simulink model "planta_PROTEC_fornalha_LC"  (Simulink 8.8)
settings: Solver=ode3  StartTime=0.0  StopTime=800  FixedStep=tempo_amostragem  MaxStep=1e1  MinStep=1e-2  EnableMultiTasking=on
InitFcn:
  | planta_PROTEC_inicializacao
values from neighbouring files (symbols this model uses):
  Estado_Estacionario = [2 38.1987406965 21.9709981215 1.00092553605 3.07737941356 1.5 0.843438999559 0.0384242731301 0.118136727311 1.3 0.304251987406 0.577644341688 ... (188 elements, 1x188)]    [planta_PROTEC_estado_estacionario_inicial.mat]
  tempo_amostragem = 1e-2    (= 0.01)    [planta_PROTEC_inicializacao.m]
libraries: simulink_extras x6
(part 3 of 3)

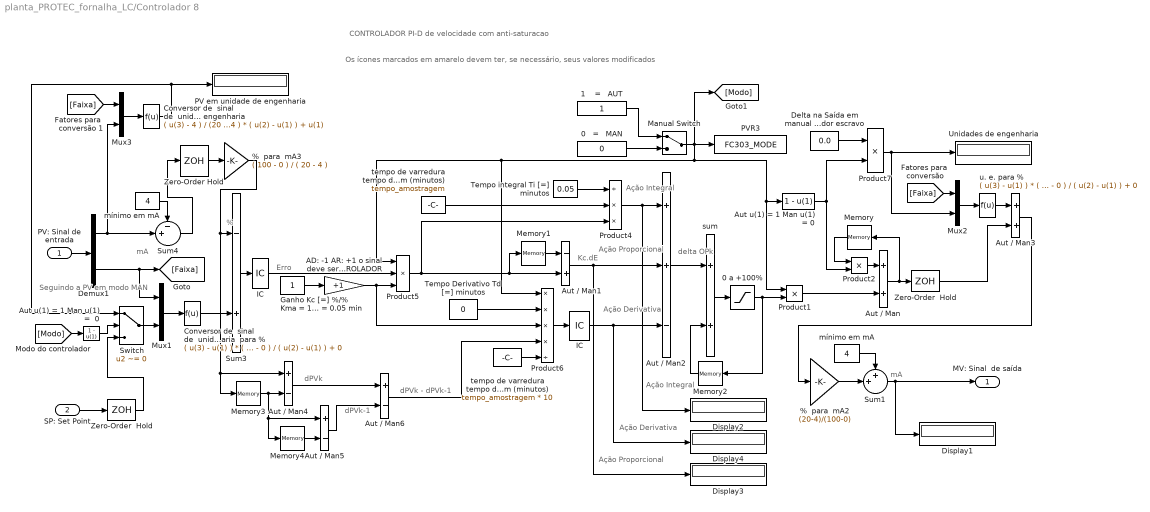
== system planta_PROTEC_fornalha_LC/Controlador 8 ==
  note: Ação
      | Derivativa
  note: dPVk - dPVk-1
  note: dPVk
  note: dPVk-1
  note: delta
      | OPk
  note: Ação
      | Integral
  note: Ação
      | Proporcional
  note: Kc.dE
  note: %
  note: mA
  note: CONTROLADOR PI-D de velocidade com anti-saturacao
  note: Os ícones marcados em amarelo devem ter, se necessário, seus valores modificados
  note: Erro
  note: mA
  note: Ação
      | Integral
  note: Ação
      | Derivativa
  note: Ação
      | Proporcional
  note: Seguindo a PV
      | em modo MAN
  PV: Sinal de entrada : Inport
  SP: Set Point : Inport  Port=2
  "  1    =   AUT" : Constant
  " IC" : InitialCondition  Value=0
  %  para  mA2 : Gain  Gain=(20-4)/(100-0)  SaturateOnIntegerOverflow=on  OutDataTypeStr=Inherit: Same as input  ParamDataTypeStr=Inherit: Same as input
  %  para  mA3 : Gain  Gain=( 100 - 0 ) / ( 20 - 4 )  SaturateOnIntegerOverflow=on  OutDataTypeStr=Inherit: Same as input  ParamDataTypeStr=Inherit: Same as input
  0   =   MAN : Constant  Value=0
  0 a +100% : Saturate  UpperLimit=100  LowerLimit=0  LinearizeAsGain=off
  "AD: -1 AR: +1 o sinal deve ser modificado para a  correta  AÇÃO  DO  CONTROLADOR  " : Gain  Gain=+1  SaturateOnIntegerOverflow=on  OutDataTypeStr=Inherit: Same as input  ParamDataTypeStr=Inherit: Same as input
  Aut / Man : Sum  SaturateOnIntegerOverflow=on  InputSameDT=on  OutDataTypeStr=Inherit: Same as first input
  Aut / Man1 : Sum  Inputs=-+  SaturateOnIntegerOverflow=on  InputSameDT=on  OutDataTypeStr=Inherit: Same as first input
  Aut / Man2 : Sum  Inputs=++-  SaturateOnIntegerOverflow=on  InputSameDT=on  OutDataTypeStr=Inherit: Same as first input
  Aut / Man3 : Sum  SaturateOnIntegerOverflow=on  InputSameDT=on  OutDataTypeStr=Inherit: Same as first input
  Aut / Man4 : Sum  Inputs=+-  SaturateOnIntegerOverflow=on  InputSameDT=on  OutDataTypeStr=Inherit: Same as first input
  Aut / Man5 : Sum  Inputs=+-  SaturateOnIntegerOverflow=on  InputSameDT=on  OutDataTypeStr=Inherit: Same as first input
  Aut / Man6 : Sum  Inputs=+-  SaturateOnIntegerOverflow=on  InputSameDT=on  OutDataTypeStr=Inherit: Same as first input
  Aut u(1) = 1 Man u(1) =  0 : Fcn  Expr=1 - u(1)
  Aut u(1) = 1 Man u(1) = 0 : Fcn  Expr=1 - u(1)
  Conversor de  sinal de  unidades  de  engenharia  para % : Fcn  Expr=( u(3) - u(1) ) * ( 100 - 0 ) / ( u(2) - u(1) ) + 0
  Conversor de  sinal de  unidades  de  mA  para  engenharia : Fcn  Expr=( u(3) - 4 ) / (20 - 4 ) * ( u(2) - u(1) ) + u(1)
  Delta na Saída em manual do controlador [=] unidades de engenharia do SP do controlador escravo : Constant  Value=0.0
  Demux1 : Demux  Outputs=[ 1 2 ]
  Display{1..4} (4 alike) : Display
  Ganho Kc [=] %/% Kma = 1 mA/mA Lambda = 0.05 min : Constant
  IC : InitialCondition  Value=0
  Manual Switch : ManualSwitch
  Memory{,2..4} (4 alike) : Memory  X0=50  InheritSampleTime=on
  Memory1 : Memory  InheritSampleTime=on
  Mux1 : Mux  Inputs=[ 2 1 ]
  Mux2 : Mux  Inputs=[ 2 1 ]
  Mux3 : Mux  Inputs=[ 2 1 ]
  PV em unidade de engenharia : Display
  PVR3 : ToWorkspace  VariableName=FC303_MODE  SampleTime=-1
      settings: Decimation=10
  Product1 : Product  SaturateOnIntegerOverflow=on  RndMeth=Zero  InputSameDT=on  OutDataTypeStr=Inherit: Same as first input
  Product2 : Product  SaturateOnIntegerOverflow=on  RndMeth=Zero  InputSameDT=on  OutDataTypeStr=Inherit: Same as first input
  Product4 : Product  Inputs=/**  SaturateOnIntegerOverflow=on  RndMeth=Zero  InputSameDT=on  OutDataTypeStr=Inherit: Same as first input
  Product5 : Product  Inputs=3  SaturateOnIntegerOverflow=on  RndMeth=Zero  InputSameDT=on  OutDataTypeStr=Inherit: Same as first input
  Product6 : Product  Inputs=****/  SaturateOnIntegerOverflow=on  RndMeth=Zero  InputSameDT=on  OutDataTypeStr=Inherit: Same as first input
  Product7 : Product  SaturateOnIntegerOverflow=on  RndMeth=Zero  InputSameDT=on  OutDataTypeStr=Inherit: Same as first input
  Sum1 : Sum  Inputs=++|  SaturateOnIntegerOverflow=on  InputSameDT=on  OutDataTypeStr=Inherit: Same as first input
  Sum3 : Sum  Inputs=-+  SaturateOnIntegerOverflow=on  InputSameDT=on  OutDataTypeStr=Inherit: Same as first input
  Sum4 : Sum  Inputs=-+|  SaturateOnIntegerOverflow=on  InputSameDT=on  OutDataTypeStr=Inherit: Same as first input
  Switch : Switch  Criteria=u2 ~= 0  RndMeth=Nearest  SaturateOnIntegerOverflow=on
  Tempo Derivativo Td [=] minutos : Constant  Value=0
  Tempo integral Ti [=] minutos : Constant  Value=0.05
  Unidades de engenharia : Display
  Zero-Order  Hold : ZeroOrderHold  SampleTime=tempo_amostragem
  "Zero-Order  Hold " : ZeroOrderHold  SampleTime=tempo_amostragem
  "Zero-Order Hold " : ZeroOrderHold  SampleTime=tempo_amostragem
  mínimo em mA : Constant  Value=4
  "mínimo em mA " : Constant  Value=4
  sum : Sum  SaturateOnIntegerOverflow=on  InputSameDT=on  OutDataTypeStr=Inherit: Same as first input
  tempo de varredura tempo de amostragem (minutos) : Constant  Value=tempo_amostragem
  "tempo de varredura tempo de amostragem (minutos) " : Constant  Value=tempo_amostragem * 10
  u. e. para % : Fcn  Expr=( u(3) - u(1) ) * ( 100 - 0 ) / ( u(2) - u(1) ) + 0
  MV: Sinal  de saída : Outport
  wires:
  "AD: -1 AR: +1 o sinal deve ser modificado para a  correta  AÇÃO  DO  CONTROLADOR  "/1 -> Product5/3, Product6/3
  " IC"/1 -> Aut / Man2/3, Display4/1
  "tempo de varredura tempo de amostragem (minutos) "/1 -> Product6/5
  Aut / Man5/1 -> Aut / Man6/2
  Aut / Man4/1 -> Aut / Man6/1
  Conversor de  sinal de  unidades  de  engenharia  para %/1 -> Sum3/2
  Product6/1 -> " IC"/1
  Tempo Derivativo Td [=] minutos/1 -> Product6/2
  Aut / Man6/1 -> Product6/4
  Memory4/1 -> Aut / Man5/2
  Memory3/1 -> Aut / Man4/2, Aut / Man5/1, Memory4/1
  Ganho Kc [=] %/% Kma = 1 mA/mA Lambda = 0.05 min/1 -> "AD: -1 AR: +1 o sinal deve ser modificado para a  correta  AÇÃO  DO  CONTROLADOR  "/1
  IC/1 -> Product5/2
  0 a +100%/1 -> Product1/2, Memory2/1
  Memory2/1 -> sum/2
  sum/1 -> 0 a +100%/1
  Aut / Man2/1 -> sum/1
  Aut / Man1/1 -> Aut / Man2/2, Display3/1
  Product4/1 -> Aut / Man2/1, Display2/1
  Memory1/1 -> Aut / Man1/1
  Memory/1 -> Product2/1
  Aut / Man/1 -> Memory/1, Zero-Order  Hold/1
  Aut u(1) = 1 Man u(1) = 0/1 -> Product2/2, Product7/2
  Product2/1 -> Aut / Man/1
  Product1/1 -> Aut / Man/2
  Product5/1 -> Memory1/1, Aut / Man1/2, Product4/3
  Sum3/1 -> IC/1
  mínimo em mA/1 -> Sum4/1
  Demux1/1 -> Sum4/2, Mux3/2
  Mux1/1 -> Conversor de  sinal de  unidades  de  engenharia  para %/1
  SP: Set Point/1 -> "Zero-Order  Hold "/1
  PV: Sinal de entrada/1 -> Demux1/1
  "mínimo em mA "/1 -> Sum1/1
  Sum1/1 -> MV: Sinal  de saída/1, Display1/1
  Sum4/1 -> "Zero-Order Hold "/1
  "Zero-Order Hold "/1 -> %  para  mA3/1
  %  para  mA3/1 -> Memory3/1, Aut / Man4/1, Sum3/1
  Manual Switch/1 -> Aut u(1) = 1 Man u(1) = 0/1, Product1/1, Product5/1, Product6/1, [Modo], PVR3/1
  Delta na Saída em manual do controlador [=] unidades de engenharia do SP do controlador escravo/1 -> Product7/1
  Product7/1 -> Unidades de engenharia/1, Mux2/2
  Demux1/2 -> Mux1/1, [Faixa]
  "Zero-Order  Hold "/1 -> Switch/3
  u. e. para %/1 -> Aut / Man3/1
  Zero-Order  Hold/1 -> Aut / Man3/2
  Mux2/1 -> u. e. para %/1
  [Faixa] -> Mux2/1
  Aut / Man3/1 -> %  para  mA2/1
  %  para  mA2/1 -> Sum1/2
  "  1    =   AUT"/1 -> Manual Switch/1
  0   =   MAN/1 -> Manual Switch/2
  [Modo] -> Aut u(1) = 1 Man u(1) =  0/1
  Switch/1 -> Mux1/2
  Aut u(1) = 1 Man u(1) =  0/1 -> Switch/2
  Mux3/1 -> Conversor de  sinal de  unidades  de  mA  para  engenharia/1
  [Faixa] -> Mux3/1
  Conversor de  sinal de  unidades  de  mA  para  engenharia/1 -> Switch/1, PV em unidade de engenharia/1
  Tempo integral Ti [=] minutos/1 -> Product4/1
  tempo de varredura tempo de amostragem (minutos)/1 -> Product4/2

== system planta_PROTEC_fornalha_LC/Dados economicos da  Planta PROTEC1 ==
  note: Sugestões e críticas enviar para o autor:
      |
      | e-mail: kalid@ufba.br
      |
      | Departamento de Engenharia Química da UFBA
      | Tel: (71) 3283.9811  ou  (71) 9188.3316
      | Arquivos e outras informações em
      |
      | www.PEI.ufba.br
  note: INFORMAÇÕES  PARA  AVALIAÇÃO  ECONÔMICA  DA  PLANTA  PROTEC
      |
      | Preço de compra de A:                   prA =   1 000.xA^8             u.e./t de A
      | Preço de venda  de B:                    prB =  10 000.xB^0.5         u.e./t de produto, para xB >= 0.755
      |                                                        prB =    1 000.xB                u.e./t de produto, para xB < 0.755
      | Preço de compra do combustível:   prC =   3 000                     u.e./t de combustível
      | Preço do tratamento do efluente:    prE =   2 000                     u.e./t de efluente
      | Preço de venda  de vapor:              prV =      500.PV^2/18.52  u.e./t de produto
      | Preço do catalisador:                   prCat = 10 000/kg de catalisador
      | Custo de processamento:                ctP =     500.(Fp)^3          u.e./t de carga processada
      | O custo de processamento inclui todos os custos variaveis, exceto os explicitados anteriormente
      |
      | xA - fração molar de A na alimentação
      | xB - fração molar de B no produto
      | PV - Pressão do Vapor [=] kgf/cm²
      | Fp - vazão processada
      |
      | u.e. - unidade econômica

== system planta_PROTEC_fornalha_LC/E 1 ==
  note: Exaustor
  Sinal de entrada : Inport
  Sinal de saída : Outport
  wires:
  Sinal de entrada/1 -> Sinal de saída/1

== system planta_PROTEC_fornalha_LC/E 312 ==
  note: Exaustor
  Sinal de entrada : Inport
  Sinal de saída : Outport
  wires:
  Sinal de entrada/1 -> Sinal de saída/1

== system planta_PROTEC_fornalha_LC/FE 1 ==
  note: Placa de orifício
  note: F
  note: T
  In1 : Inport
  Demux26 : Demux  Outputs=2
  Terminator1 : Terminator
  Out1 : Outport
  Out2 : Outport  Port=2
  wires:
  Demux26/2 -> Terminator1/1
  Demux26/1 -> Out1/1
  In1/1 -> Demux26/1, Out2/1

== system planta_PROTEC_fornalha_LC/FE 2 ==
  note: x
  note: T
  note: F
  note: Placa de orifício
  In1 : Inport
  Demux26 : Demux  Outputs=3
  Terminator1 : Terminator
  Terminator9 : Terminator
  Out1 : Outport
  Out2 : Outport  Port=2
  wires:
  In1/1 -> Out2/1, Demux26/1
  Demux26/1 -> Out1/1
  Demux26/3 -> Terminator9/1
  Demux26/2 -> Terminator1/1

== system planta_PROTEC_fornalha_LC/FE 302 ==
  note: T
  note: F
  note: Placa de orifício
  In1 : Inport
  Demux26 : Demux  Outputs=2
  Terminator1 : Terminator
  Out1 : Outport
  Out2 : Outport  Port=2
  wires:
  In1/1 -> Out2/1, Demux26/1
  Demux26/1 -> Out1/1
  Demux26/2 -> Terminator1/1

== system planta_PROTEC_fornalha_LC/FE 303 ==
  note: Placa de orifício
  note: F
  note: T
  note: x
  In1 : Inport
  Demux26 : Demux  Outputs=3
  Terminator1 : Terminator
  Terminator9 : Terminator
  Out1 : Outport
  Out2 : Outport  Port=2
  wires:
  Demux26/2 -> Terminator1/1
  Demux26/3 -> Terminator9/1
  Demux26/1 -> Out1/1
  In1/1 -> Demux26/1, Out2/1

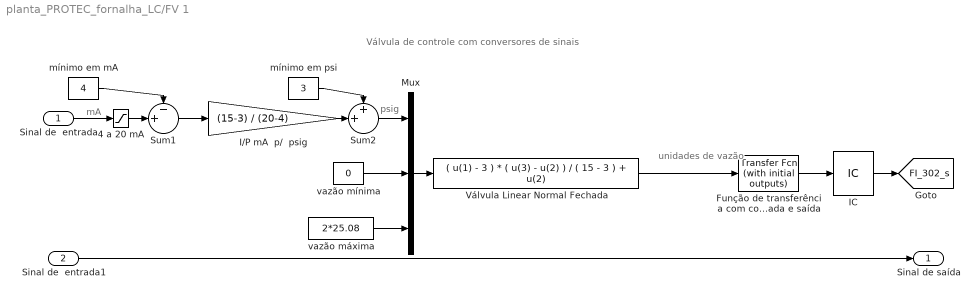
== system planta_PROTEC_fornalha_LC/FV 1 ==
  note: mA
  note: Válvula de controle com conversores de sinais
  note: unidades
      | de vazão
  note: psig
  Sinal de  entrada : Inport
  Sinal de  entrada1 : Inport  Port=2
  4 a 20 mA : Saturate  UpperLimit=20  LowerLimit=4
  Função de transferência com condição inicial  na entrada e saída : simulink_extras/Additional Linear/Transfer Fcn (with initial outputs)  N=[1]  D="[0.05   1 ]"  Y0=Estado_Estacionario(38)  U0=Estado_Estacionario(38)
  I/P mA  p/  psig : Gain  Gain=(15-3) / (20-4)  SaturateOnIntegerOverflow=on  OutDataTypeStr=Inherit: Same as input  ParamDataTypeStr=Inherit: Same as input
  IC : InitialCondition  Value=25.08
  Mux : Mux  Inputs=3
  Sum1 : Sum  Inputs=-+|  SaturateOnIntegerOverflow=on  InputSameDT=on  OutDataTypeStr=Inherit: Same as first input
  Sum2 : Sum  Inputs=++|  SaturateOnIntegerOverflow=on  InputSameDT=on  OutDataTypeStr=Inherit: Same as first input
  Válvula Linear Normal Fechada : Fcn  Expr=( u(1) - 3 ) * ( u(3) - u(2) ) / ( 15 - 3 ) + u(2)
  mínimo em mA : Constant  Value=4
  mínimo em psi : Constant  Value=3
  vazão máxima : Constant  Value=2*25.08
  vazão mínima : Constant  Value=0
  Sinal de saída : Outport
  tag scope: FI_302_s=global
  wires:
  vazão máxima/1 -> Mux/3
  vazão mínima/1 -> Mux/2
  Mux/1 -> Válvula Linear Normal Fechada/1
  mínimo em mA/1 -> Sum1/1
  Sum1/1 -> I/P mA  p/  psig/1
  Sinal de  entrada/1 -> 4 a 20 mA/1
  I/P mA  p/  psig/1 -> Sum2/2
  Sum2/1 -> Mux/1
  mínimo em psi/1 -> Sum2/1
  Válvula Linear Normal Fechada/1 -> Função de transferência com condição inicial  na entrada e saída/1
  Função de transferência com condição inicial  na entrada e saída/1 -> IC/1
  Sinal de  entrada1/1 -> Sinal de saída/1
  IC/1 -> [FI_302_s]
  4 a 20 mA/1 -> Sum1/2

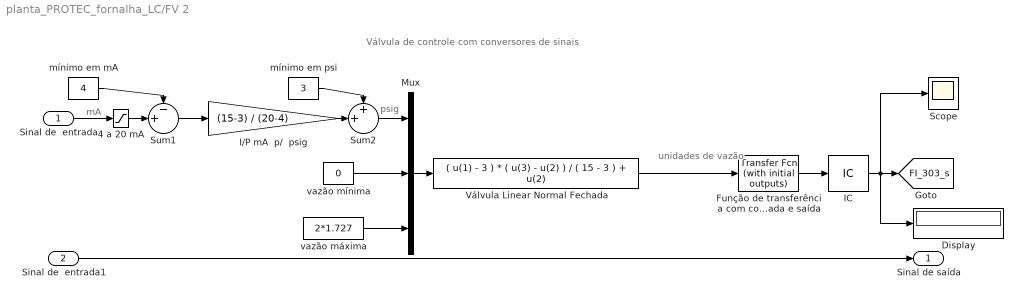
== system planta_PROTEC_fornalha_LC/FV 2 ==
  note: psig
  note: unidades
      | de vazão
  note: Válvula de controle com conversores de sinais
  note: mA
  Sinal de  entrada : Inport
  Sinal de  entrada1 : Inport  Port=2
  4 a 20 mA : Saturate  UpperLimit=20  LowerLimit=4
  Display : Display
  Função de transferência com condição inicial  na entrada e saída : simulink_extras/Additional Linear/Transfer Fcn (with initial outputs)  N=[1]  D="[ 0.05   1 ]"  Y0=Estado_Estacionario(39)  U0=Estado_Estacionario(39)
  I/P mA  p/  psig : Gain  Gain=(15-3) / (20-4)  SaturateOnIntegerOverflow=on  OutDataTypeStr=Inherit: Same as input  ParamDataTypeStr=Inherit: Same as input
  IC : InitialCondition  Value=1.727
  Mux : Mux  Inputs=3
  Scope : Scope
  Sum1 : Sum  Inputs=-+|  SaturateOnIntegerOverflow=on  InputSameDT=on  OutDataTypeStr=Inherit: Same as first input
  Sum2 : Sum  Inputs=++|  SaturateOnIntegerOverflow=on  InputSameDT=on  OutDataTypeStr=Inherit: Same as first input
  Válvula Linear Normal Fechada : Fcn  Expr=( u(1) - 3 ) * ( u(3) - u(2) ) / ( 15 - 3 ) + u(2)
  mínimo em mA : Constant  Value=4
  mínimo em psi : Constant  Value=3
  vazão máxima : Constant  Value=2*1.727
  vazão mínima : Constant  Value=0
  Sinal de saída : Outport
  tag scope: FI_303_s=global
  wires:
  4 a 20 mA/1 -> Sum1/2
  IC/1 -> [FI_303_s], Scope/1, Display/1
  Sinal de  entrada1/1 -> Sinal de saída/1
  Função de transferência com condição inicial  na entrada e saída/1 -> IC/1
  Válvula Linear Normal Fechada/1 -> Função de transferência com condição inicial  na entrada e saída/1
  mínimo em psi/1 -> Sum2/1
  Sum2/1 -> Mux/1
  I/P mA  p/  psig/1 -> Sum2/2
  Sinal de  entrada/1 -> 4 a 20 mA/1
  Sum1/1 -> I/P mA  p/  psig/1
  mínimo em mA/1 -> Sum1/1
  Mux/1 -> Válvula Linear Normal Fechada/1
  vazão mínima/1 -> Mux/2
  vazão máxima/1 -> Mux/3

== system planta_PROTEC_fornalha_LC/FV 302 ==
  note: psig
  note: unidades
      | de vazão
  note: Válvula de controle com conversores de sinais
  note: mA
  Sinal de  entrada : Inport
  Sinal de  entrada1 : Inport  Port=2
  4 a 20 mA : Saturate  UpperLimit=20  LowerLimit=4
  Função de transferência com condição inicial  na entrada e saída : simulink_extras/Additional Linear/Transfer Fcn (with initial outputs)  N=[1]  D="[0.05   1 ]"  Y0=Estado_Estacionario(38)  U0=Estado_Estacionario(38)
  I/P mA  p/  psig : Gain  Gain=(15-3) / (20-4)  SaturateOnIntegerOverflow=on  OutDataTypeStr=Inherit: Same as input  ParamDataTypeStr=Inherit: Same as input
  IC : InitialCondition  Value=25.08
  Mux : Mux  Inputs=3
  Sum1 : Sum  Inputs=-+|  SaturateOnIntegerOverflow=on  InputSameDT=on  OutDataTypeStr=Inherit: Same as first input
  Sum2 : Sum  Inputs=++|  SaturateOnIntegerOverflow=on  InputSameDT=on  OutDataTypeStr=Inherit: Same as first input
  Válvula Linear Normal Fechada : Fcn  Expr=( u(1) - 3 ) * ( u(3) - u(2) ) / ( 15 - 3 ) + u(2)
  mínimo em mA : Constant  Value=4
  mínimo em psi : Constant  Value=3
  vazão máxima : Constant  Value=2*25.08
  vazão mínima : Constant  Value=0
  Sinal de saída : Outport
  tag scope: FI_302=global
  wires:
  4 a 20 mA/1 -> Sum1/2
  IC/1 -> [FI_302]
  Sinal de  entrada1/1 -> Sinal de saída/1
  Função de transferência com condição inicial  na entrada e saída/1 -> IC/1
  Válvula Linear Normal Fechada/1 -> Função de transferência com condição inicial  na entrada e saída/1
  mínimo em psi/1 -> Sum2/1
  Sum2/1 -> Mux/1
  I/P mA  p/  psig/1 -> Sum2/2
  Sinal de  entrada/1 -> 4 a 20 mA/1
  Sum1/1 -> I/P mA  p/  psig/1
  mínimo em mA/1 -> Sum1/1
  Mux/1 -> Válvula Linear Normal Fechada/1
  vazão mínima/1 -> Mux/2
  vazão máxima/1 -> Mux/3

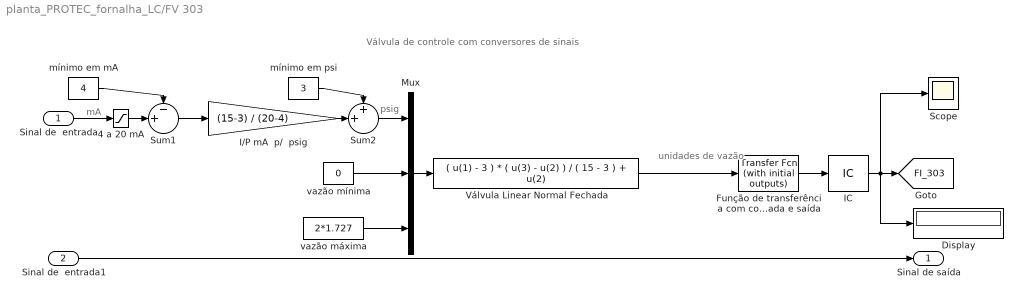
== system planta_PROTEC_fornalha_LC/FV 303 ==
  note: mA
  note: Válvula de controle com conversores de sinais
  note: unidades
      | de vazão
  note: psig
  Sinal de  entrada : Inport
  Sinal de  entrada1 : Inport  Port=2
  4 a 20 mA : Saturate  UpperLimit=20  LowerLimit=4
  Display : Display
  Função de transferência com condição inicial  na entrada e saída : simulink_extras/Additional Linear/Transfer Fcn (with initial outputs)  N=[1]  D="[ 0.05   1 ]"  Y0=Estado_Estacionario(39)  U0=Estado_Estacionario(39)
  I/P mA  p/  psig : Gain  Gain=(15-3) / (20-4)  SaturateOnIntegerOverflow=on  OutDataTypeStr=Inherit: Same as input  ParamDataTypeStr=Inherit: Same as input
  IC : InitialCondition  Value=1.727
  Mux : Mux  Inputs=3
  Scope : Scope
  Sum1 : Sum  Inputs=-+|  SaturateOnIntegerOverflow=on  InputSameDT=on  OutDataTypeStr=Inherit: Same as first input
  Sum2 : Sum  Inputs=++|  SaturateOnIntegerOverflow=on  InputSameDT=on  OutDataTypeStr=Inherit: Same as first input
  Válvula Linear Normal Fechada : Fcn  Expr=( u(1) - 3 ) * ( u(3) - u(2) ) / ( 15 - 3 ) + u(2)
  mínimo em mA : Constant  Value=4
  mínimo em psi : Constant  Value=3
  vazão máxima : Constant  Value=2*1.727
  vazão mínima : Constant  Value=0
  Sinal de saída : Outport
  tag scope: FI_303=global
  wires:
  vazão máxima/1 -> Mux/3
  vazão mínima/1 -> Mux/2
  Mux/1 -> Válvula Linear Normal Fechada/1
  mínimo em mA/1 -> Sum1/1
  Sum1/1 -> I/P mA  p/  psig/1
  Sinal de  entrada/1 -> 4 a 20 mA/1
  I/P mA  p/  psig/1 -> Sum2/2
  Sum2/1 -> Mux/1
  mínimo em psi/1 -> Sum2/1
  Válvula Linear Normal Fechada/1 -> Função de transferência com condição inicial  na entrada e saída/1
  Função de transferência com condição inicial  na entrada e saída/1 -> IC/1
  Sinal de  entrada1/1 -> Sinal de saída/1
  IC/1 -> Display/1, Scope/1, [FI_303]
  4 a 20 mA/1 -> Sum1/2

== system planta_PROTEC_fornalha_LC/Load Data1 ==

== system planta_PROTEC_fornalha_LC/Load Data2 ==

== system planta_PROTEC_fornalha_LC/Objetivos e restrições da  Planta PROTEC ==
  note: Sugestões e críticas enviar para o autor:
      | e-mail: kalid@ufba.br
      | Programa de Engenharia Industrial da UFBA
      | Tel: (71) 3283.9811  ou  (71) 9188.3316
      | Arquivos e outras informações em
      | www.PEI.ufba.br
  note: Área 100: Tanque de carga
      |
      | a) Nível máximo 3 metros.
      | b) Nível mínimo 1 metro.
      | c) Vazão de make-up máxima de  3,0 m³/min.
      | d) Vazão de make-up mínima de  0,0 m³/min.
      | e) Temperatura de descarga > 35 ºC.
  note: Área 500: Coluna de Destilação
      |
      | a) Fração molar do topo:   xBtopo   > 0,745.
      | b) Fração molar do fundo: xBfundo < 0,30.
      | c) Temperatura da alimentação entre 30 e 50 ºC.
      | d) Nível do tambor de refluxo: entre 0,5 e 1,5 metros.
      | e) Nível do fundo da coluna: entre 0,5 e 1,5 metros.
      | Obs.: condensador total, destilado saturado, pressão constante.
  note: Área 400: Reator CSTR
      |
      | a) Nível máximo 1,2 metros.
      | b) Nível mínimo  0,8 metros.
      | c) Vazão de catalisador entre 0 e 2 kg/min.
  note: Área 200: Permutador de calor
      |
      | a) Todas as Temperaturas < 60 ºC.
  note: Área 300: Fornalha
      |
      | a) Conc. O2 gases de exaustão > 0,5 mol/m³.
      | b) Temp. na saída da fornalha (processo) > 370 ºC
      | c) Temp. na saída da fornalha (processo) < 390 ºC.
      | d) Temp. dos gases de exaustão < 1000 ºC.
  note: Objetivos operacionais:    a) Operar de forma estável e suave.
      |                                              b) A planta deve operar nas condições abaixo quando a carga aumenta em 15% e quando diminui em 30%.
      |                                              c) O custo operacional deve ser SEMPRE minimizado.
      |                                              d) Todas as restrições abaixo devem ser RIGOROSAMENTE obedecidas.
  note: Válvulas
      |
      | a) Operar entre 15 e 85 % de abertura.
  note: Área 700: Caldeira
      |
      | a) Nível máximo  + 50 mm.
      | b) Nível mínimo    - 50 mm.
      | c) Pressão do vapor entre 17 e 19 kgf/cm².
      | d) Conc. O2 gases de exaustão > 0,5 mol/m³.
  note: Área 900: Tratamento de efluente
      |
      | a) Vazão de efluente < 0,35  m³/min.
      | b) Nível tanque de efluente < 1,8 m.
  note: Área 600: Válvula de 4 vias
      |
      |         Não há restrições.
  note: Área 800: Header de vapor
      |
      |         Não há restrições.

== system planta_PROTEC_fornalha_LC/Transmissor 1 ==
  note: Transmissor
  note: mA
  Sinal de entrada unidades de engenharia : Inport
  Memory4 : Memory  X0=25.08
  Mux : Mux  Inputs=3
  Mux1 : Mux  Inputs=3
  PV máximo : Constant  Value=2*25.08
  PV mínimo : Constant  Value=0
  Transmissor : Fcn  Expr=( u(1) - u(2) ) * ( 20 - 4) / ( u(3) - u(2) ) + 4
  Sinal de saída : Outport
  wires:
  Mux1/1 -> Sinal de saída/1
  Transmissor/1 -> Mux1/1
  Sinal de entrada unidades de engenharia/1 -> Memory4/1
  PV máximo/1 -> Mux1/3, Mux/3
  PV mínimo/1 -> Mux1/2, Mux/2
  Mux/1 -> Transmissor/1
  Memory4/1 -> Mux/1

== system planta_PROTEC_fornalha_LC/Transmissor 2 ==
  note: Transmissor
  note: mA
  Sinal de entrada unidades de engenharia : Inport
  Memory4 : Memory  X0=1.727
  Mux : Mux  Inputs=3
  Mux1 : Mux  Inputs=3
  PV máximo : Constant  Value=2*1.727
  PV mínimo : Constant  Value=0
  Transmissor : Fcn  Expr=( u(1) - u(2) ) * ( 20 - 4) / ( u(3) - u(2) ) + 4
  Sinal de saída : Outport
  wires:
  Mux1/1 -> Sinal de saída/1
  Transmissor/1 -> Mux1/1
  Sinal de entrada unidades de engenharia/1 -> Memory4/1
  PV máximo/1 -> Mux1/3, Mux/3
  PV mínimo/1 -> Mux1/2, Mux/2
  Mux/1 -> Transmissor/1
  Memory4/1 -> Mux/1

== system planta_PROTEC_fornalha_LC/Transmissor 3 ==
  note: Transmissor
  note: mA
  Sinal de entrada unidades de engenharia : Inport
  Memory4 : Memory  X0=384.0986
  Mux : Mux  Inputs=3
  Mux1 : Mux  Inputs=3
  PV máximo : Constant  Value=384*2
  PV mínimo : Constant  Value=0
  Transmissor : Fcn  Expr=( u(1) - u(2) ) * ( 20 - 4) / ( u(3) - u(2) ) + 4
  Sinal de saída : Outport
  wires:
  Mux1/1 -> Sinal de saída/1
  Transmissor/1 -> Mux1/1
  Sinal de entrada unidades de engenharia/1 -> Memory4/1
  PV máximo/1 -> Mux1/3, Mux/3
  PV mínimo/1 -> Mux1/2, Mux/2
  Mux/1 -> Transmissor/1
  Memory4/1 -> Mux/1

== system planta_PROTEC_fornalha_LC/Transmissor 4 ==
  note: mA
  note: Transmissor
  Sinal de entrada unidades de engenharia : Inport
  Memory4 : Memory  X0=25.08
  Mux : Mux  Inputs=3
  Mux1 : Mux  Inputs=3
  PV máximo : Constant  Value=2*25.08
  PV mínimo : Constant  Value=0
  Transmissor : Fcn  Expr=( u(1) - u(2) ) * ( 20 - 4) / ( u(3) - u(2) ) + 4
  Sinal de saída : Outport
  wires:
  Memory4/1 -> Mux/1
  Mux/1 -> Transmissor/1
  PV mínimo/1 -> Mux/2, Mux1/2
  PV máximo/1 -> Mux/3, Mux1/3
  Sinal de entrada unidades de engenharia/1 -> Memory4/1
  Transmissor/1 -> Mux1/1
  Mux1/1 -> Sinal de saída/1

== system planta_PROTEC_fornalha_LC/Transmissor 5 ==
  note: mA
  note: Transmissor
  Sinal de entrada unidades de engenharia : Inport
  Memory4 : Memory  X0=1.727
  Mux : Mux  Inputs=3
  Mux1 : Mux  Inputs=3
  PV máximo : Constant  Value=2*1.727
  PV mínimo : Constant  Value=0
  Transmissor : Fcn  Expr=( u(1) - u(2) ) * ( 20 - 4) / ( u(3) - u(2) ) + 4
  Sinal de saída : Outport
  wires:
  Memory4/1 -> Mux/1
  Mux/1 -> Transmissor/1
  PV mínimo/1 -> Mux/2, Mux1/2
  PV máximo/1 -> Mux/3, Mux1/3
  Sinal de entrada unidades de engenharia/1 -> Memory4/1
  Transmissor/1 -> Mux1/1
  Mux1/1 -> Sinal de saída/1

== system planta_PROTEC_fornalha_LC/Transmissor 6 ==
  note: mA
  note: Transmissor
  Sinal de entrada unidades de engenharia : Inport
  Memory4 : Memory  X0=384.0986
  Mux : Mux  Inputs=3
  Mux1 : Mux  Inputs=3
  PV máximo : Constant  Value=384*2
  PV mínimo : Constant  Value=0
  Transmissor : Fcn  Expr=( u(1) - u(2) ) * ( 20 - 4) / ( u(3) - u(2) ) + 4
  Sinal de saída : Outport
  wires:
  Memory4/1 -> Mux/1
  Mux/1 -> Transmissor/1
  PV mínimo/1 -> Mux/2, Mux1/2
  PV máximo/1 -> Mux/3, Mux1/3
  Sinal de entrada unidades de engenharia/1 -> Memory4/1
  Transmissor/1 -> Mux1/1
  Mux1/1 -> Sinal de saída/1

== system planta_PROTEC_fornalha_LC/V 1 ==
  note: Ventilador
  Sinal de entrada : Inport
  Sinal de saída : Outport
  wires:
  Sinal de entrada/1 -> Sinal de saída/1

== system planta_PROTEC_fornalha_LC/V 302 ==
  note: Ventilador
  Sinal de entrada : Inport
  Sinal de saída : Outport
  wires:
  Sinal de entrada/1 -> Sinal de saída/1

== system planta_PROTEC_fornalha_LC/t/min ==
  note: mA
  In1 : Inport
  Conversor de  sinal de  unidades  de  mA  para  engenharia2 : Fcn  Expr=( u(3) - 4 ) / (20 - 4 ) * ( u(2) - u(1) ) + u(1)
  Demux1 : Demux  Outputs=[ 1 2 ]
  Mux3 : Mux  Inputs=[ 2 1 ]
  Out1 : Outport
  wires:
  Conversor de  sinal de  unidades  de  mA  para  engenharia2/1 -> Out1/1
  [Faixa] -> Mux3/1
  Mux3/1 -> Conversor de  sinal de  unidades  de  mA  para  engenharia2/1
  Demux1/2 -> [Faixa]
  In1/1 -> Demux1/1
  Demux1/1 -> Mux3/2

== system planta_PROTEC_fornalha_LC/t/min1 ==
  note: mA
  In1 : Inport
  Conversor de  sinal de  unidades  de  mA  para  engenharia2 : Fcn  Expr=( u(3) - 4 ) / (20 - 4 ) * ( u(2) - u(1) ) + u(1)
  Demux1 : Demux  Outputs=[ 1 2 ]
  Mux3 : Mux  Inputs=[ 2 1 ]
  Out1 : Outport
  wires:
  Demux1/1 -> Mux3/2
  In1/1 -> Demux1/1
  Demux1/2 -> [Faixa]
  Mux3/1 -> Conversor de  sinal de  unidades  de  mA  para  engenharia2/1
  [Faixa] -> Mux3/1
  Conversor de  sinal de  unidades  de  mA  para  engenharia2/1 -> Out1/1

== system planta_PROTEC_fornalha_LC/u.e.1 ==
  note: mA
  In1 : Inport
  Conversor de  sinal de  unidades  de  mA  para  engenharia2 : Fcn  Expr=( u(3) - 4 ) / (20 - 4 ) * ( u(2) - u(1) ) + u(1)  SampleTime=tempo_amostragem
  Demux1 : Demux  Outputs=[ 1 2 ]
  Mux3 : Mux  Inputs=[ 2 1 ]
  Out1 : Outport
  wires:
  Conversor de  sinal de  unidades  de  mA  para  engenharia2/1 -> Out1/1
  [Faixa] -> Mux3/1
  Mux3/1 -> Conversor de  sinal de  unidades  de  mA  para  engenharia2/1
  Demux1/2 -> [Faixa]
  In1/1 -> Demux1/1
  Demux1/1 -> Mux3/2

== system planta_PROTEC_fornalha_LC/300: FORNALHA/Tempo Morto nos tubos ==
  note: Tempo morto devido a distância entre os equipamentos
  F,xA,xB,xC : Inport
  Demux6 : Demux  Outputs=[1 3]
  Product : Product  Inputs=*/  SaturateOnIntegerOverflow=on  RndMeth=Zero  InputSameDT=on  OutDataTypeStr=Inherit: Same as first input
  Variable Transport Delay : VariableTransportDelay  MaximumDelay=100  InitialOutput=[ Estado_Estacionario(7:9) ]  MaximumPoints=16384
  Volume dos tubos [=] m³ : Constant  Value=4
  "xA,xB, xC" : Outport
  wires:
  Product/1 -> Variable Transport Delay/2
  Volume dos tubos [=] m³/1 -> Product/1
  Demux6/2 -> Variable Transport Delay/1
  Variable Transport Delay/1 -> "xA,xB, xC"/1
  Demux6/1 -> Product/2
  F,xA,xB,xC/1 -> Demux6/1

== system planta_PROTEC_fornalha_LC/300: FORNALHA1/Tempo Morto nos tubos ==
  note: Tempo morto devido a distância entre os equipamentos
  F,xA,xB,xC : Inport
  Demux6 : Demux  Outputs=[1 3]
  Product : Product  Inputs=*/  SaturateOnIntegerOverflow=on  RndMeth=Zero  InputSameDT=on  OutDataTypeStr=Inherit: Same as first input
  Variable Transport Delay : VariableTransportDelay  MaximumDelay=100  InitialOutput=[ Estado_Estacionario(7:9) ]  MaximumPoints=16384
  Volume dos tubos [=] m³ : Constant  Value=4
  "xA,xB, xC" : Outport
  wires:
  F,xA,xB,xC/1 -> Demux6/1
  Demux6/1 -> Product/2
  Variable Transport Delay/1 -> "xA,xB, xC"/1
  Demux6/2 -> Variable Transport Delay/1
  Volume dos tubos [=] m³/1 -> Product/1
  Product/1 -> Variable Transport Delay/2
